simulink model "ADCS_Software_v1"  (R2026a)
settings: Solver=FixedStepAuto  StopTime=Inf  FixedStep=0.05  MaxStep=0.1
model workspace (MAT data in the model file):
  I_RW : Simulink.Parameter (value not decoded)
  Sig : Simulink.Signal (value not decoded)
  h_max : Simulink.Parameter (value not decoded)
  k_desat : Simulink.Parameter (value not decoded)
  kd_detumble : Simulink.Parameter (value not decoded)
  kd_hold : Simulink.Parameter (value not decoded)
  kd_point : Simulink.Parameter (value not decoded)
  kd_slew_fast : Simulink.Parameter (value not decoded)
  kd_slew_slow : Simulink.Parameter (value not decoded)
  kd_spin : Simulink.Parameter (value not decoded)
  kp_hold : Simulink.Parameter (value not decoded)
  kp_point : Simulink.Parameter (value not decoded)
  kp_slew_fast : Simulink.Parameter (value not decoded)
  kp_slew_slow : Simulink.Parameter (value not decoded)
  kp_spin : Simulink.Parameter (value not decoded)
values from neighbouring files (symbols this model uses):
  h_max = 1.47    [parameters.m]
  I_RW = 1    [parameters.m]
  k_desat = 1    [parameters.m]
  kd_detumble = 1    [parameters.m]
  kd_point = 20    [parameters.m]
  kd_spin = 0    [parameters.m]
  kp_point = 2    [parameters.m]
  kp_spin = 1    [parameters.m]
  omega_thr = 0.1    [parameters.m]
  omega_zero = 0.01    [parameters.m]
libraries: matrix_library x10, simulink x4, aerolibutil x2
(part 2 of 2)

== matlab function ADCS_Software_v1/Subsystem3/Controller/Control Algorithms/RW Torque Commands/OPTICAL/MATLAB Function2 ==
  data: y_cm output; x_cm output; u input
function [y_cm,x_cm] = fcn(u)
% u(u>5) = uint8(255);
% y = zeros(size(u,1),size(u,2));
% for i = 1:size(u,1)
%     for j = 1:size(u,2)
%         y(i,j) = double(max(u(i,j,:)));
%     end
% end
% S = sum(sum(y));
% if S == 0
%     x_cm = 0;
%     y_cm = 0;
% else
%     x_cm = sum(sum(y.*(1:size(y,2)),2))/S - size(y,2)/2;
%     y_cm = sum(sum(y.*(1:size(y,1))',1))/S- size(y,1)/2;
% end

y = double(max(u, [], 3));

% Binary foreground
bw = y > 5;

% Connected components
CC = bwconncomp(bw, 8);

if CC.NumObjects == 0
    x_cm = 0;
    y_cm = 0;
else
    % Calculate area of every component
    areas = cellfun(@numel, CC.PixelIdxList);

    % Largest connected component = satellite
    [~, idx] = max(areas);

    satelliteMask = false(size(bw));
    satelliteMask(CC.PixelIdxList{idx}) = true;

    % Geometric centroid
    [r, c] = find(satelliteMask);

    x_cm = mean(c) - size(y,2)/2;
    y_cm = mean(r) - size(y,1)/2;
end

== matlab function ADCS_Software_v1/MATLAB Function ==
  data: image input; quaternion output; use_previous input; previous_quaternion input; attitude_deg output; valid output; info output
function [quaternion, attitude_deg, valid, info] = startracker_sl(image, use_previous, previous_quaternion)
%#codegen
%STARTRACKER_SL  startracker.m for a Simulink MATLAB Function block / C code.
%
%   [q, attitude_deg, valid, info] = STARTRACKER_SL(image, use_previous, previous_quaternion)
%
%   Same algorithm, catalogue and conventions as startracker.m, rewritten so
%   MATLAB Coder / Simulink Coder can generate C from it:
%
%     * the catalogue comes from catalogue.mat through coder.load, so it is
%       compiled into the C code as constant data -- no file I/O at run time.
%       Make catalogue.mat with convert_catalogue.m and keep it on the MATLAB
%       path (or in the model's folder) when the model is built.
%     * every array has a fixed size: no growing arrays, cells, strings,
%       graph/conncomp, accumarray, sortrows, unique, intersect or eig.
%     * the info struct is replaced by a fixed 1x8 numeric vector.
%
%   Inputs:
%
%     image                2-D uint8 frame (1024x1024 for the shipped camera).
%                          Must be fixed-size in the Simulink block.
%     use_previous         0 = lost in space, 1 = tracking around input 3
%     previous_quaternion  1x4 or 4x1 [w x y z], scalar-first, the previous
%                          boresight (camera) attitude -- e.g. the fed-back
%                          output of this block
%
%   Outputs:
%
%     quaternion    1x4 [w x y z], scalar-first, the boresight (camera)
%                   attitude [CN]: the rotation carrying inertial (J2000)
%                   components into camera components, with +Z_C the
%                   boresight, +X_C image columns, +Y_C image rows.  NaN when
%                   not solved.
%     attitude_deg  1x3 boresight RA, Dec and roll about the boresight, in
%                   degrees (roll 0 = celestial north toward image row 0).
%                   NaN when not solved.
%     valid         true when quaternion is a fix
%     info          1x8 double:
%                     1  mode            0 = lost in space, 1 = tracking
%                     2  nDetections     stars detected in the frame
%                     3  nConsidered     brightest detections used (<= 15)
%                     4  nMatched        stars used in the final QUEST
%                     5  nSearched       catalogue stars searched
%                     6  residualArcsec  mean residual, NaN when not solved
%                     7  reasonCode      0 solved
%                                        1 too few detections
%                                        2 fewer than four detections
%                                        3 triad budget exhausted
%                                        4 no confirmed pyramid
%                     8  fallbackCode    0 none
%                                        1 previous quaternion not finite / zero
%                                        2 tracking found no match
%                                        3 previous boresight in no region
%
%   VALID = FALSE IS AN ANSWER: hold the last good attitude when it is false.
%
%   In the MATLAB Function block just call this function:
%
%       function [q, att, valid, info] = fcn(image, use_previous, previous_q)
%       [q, att, valid, info] = startracker_sl(image, use_previous, previous_q);
%
%   or paste this whole file into the block (rename the first function to
%   fcn, or keep its name -- the block uses the first function).

q_BC  = [0, 0, 0.707106781186548, 0.707106781186548];   % camera mounting (from DCM_CB')
q_sky = [0.707106781186548, 0, 0, 0.707106781186548];   % Vizard sky offset (from R_sky) - SIM ONLY


% In generated code (Simulink, C) coder.load runs at compile time: the
% catalogue becomes static const data, nothing is loaded at run time.  Run as
% plain MATLAB, coder.load would read the file on every call, so it is cached.
if coder.target('MATLAB')
    catalog = cachedCatalogue();
else
    catalog = coder.load('catalogue.mat');
end

% Settings, identical to startracker.m.
kDetections = 15;        % brightest detections handed to identification
minMatched = 4;          % fewest correspondences worth a quaternion
maxTriads = 400;         % triad budget before giving up
expandRadiusPx = 3.0;    % match growth radius
trackRings = 1;          % how far the tracking region walk spreads

quaternion = NaN(1, 4);
attitude_deg = NaN(1, 3);
valid = false;
info = zeros(1, 8);
info(6) = NaN;

tolerance = 3.5 * sqrt(2) * catalog.centroidSigmaPx / catalog.focalLengthPx;

% ---------------------------------------------------------------- detect ---
if isa(image, 'uint8')
    frame = image;
else
    frame = uint8(image);
end
[u, v, nTop, nDetections] = detectStars(frame, catalog.detectionSigma, kDetections);
info(2) = nDetections;

if nDetections < minMatched
    info(7) = 1;
    return;
end

n = nTop;
body = pixelToCamera(catalog, u, v, n);   % kDetections x 3, rows 1..n valid
info(3) = n;

% -------------------------------------------------------------- identify ---
priorMask = false(size(catalog.regionCentres, 1), 1);
havePrior = false;
if use_previous ~= 0
    qPrev = double(previous_quaternion(:)');
    if ~all(isfinite(qPrev)) || norm(qPrev) == 0
        info(8) = 1;
    else
        previousDcm = quatToDcm(qPrev);
        [priorMask, nPrior] = regionsContaining(catalog, previousDcm(3, :), priorMask, false);
        if nPrior > 0
            havePrior = true;
        else
            info(8) = 3;
        end
    end
end

tracking = false;
success = false;
detectionIndex = zeros(1, 4);
catalogueIndex = zeros(1, 4);
reasonCode = 4;

if havePrior
    searchRegions = regionNeighbourhood(catalog, priorMask, trackRings);
    starMask = subsetMask(catalog, searchRegions);
    [success, detectionIndex, catalogueIndex, reasonCode] = ...
        identifyPyramid(body, n, catalog, tolerance, maxTriads, starMask);
    if success
        tracking = true;
        info(1) = 1;
        info(5) = sum(starMask);
    else
        info(8) = 2;
    end
end

if ~success
    starMask = true(size(catalog.vectors, 1), 1);       % whole catalogue
    [success, detectionIndex, catalogueIndex, reasonCode] = ...
        identifyPyramid(body, n, catalog, tolerance, maxTriads, starMask);
    info(1) = 0;
    info(5) = catalog.nStars;
end

info(7) = reasonCode;
if ~success
    return;
end

% ---------------------------------------------------------------- attitude -
% Provisional attitude from the confirmed pyramid, then grow the match set.
provisional = quatToDcm(questQuaternion(body, detectionIndex, ...
                                        catalog.vectors, catalogueIndex, 4));

poolMask = true(size(catalog.vectors, 1), 1);
if tracking
    [regionIds, ~] = regionsContaining(catalog, provisional(3, :), priorMask, true);
    poolMask = subsetMask(catalog, regionNeighbourhood(catalog, regionIds, 1));
    if ~any(poolMask)
        poolMask(:) = true;   % startracker.m: empty candidates = whole catalogue
    end
end

expandTolerance = expandRadiusPx / catalog.focalLengthPx;
[expDet, expCat, nExp] = expandMatches(provisional, body, n, catalog, ...
                                       expandTolerance, poolMask);

if nExp >= minMatched
    matchedDet = expDet;
    matchedCat = expCat;
    nMatched = nExp;
else
    matchedDet = zeros(kDetections, 1);
    matchedCat = zeros(kDetections, 1);
    matchedDet(1:4) = detectionIndex;
    matchedCat(1:4) = catalogueIndex;
    nMatched = 4;
end

q = questQuaternion(body, matchedDet, catalog.vectors, matchedCat, nMatched);
q = quatmultiply(q_sky,quatmultiply(q,q_BC));
dcm = quatToDcm(q);
[ra, dec, roll] = dcmToRadecRoll(dcm);
residualSum = 0;
for m = 1:nMatched
    b = body(matchedDet(m), :);
    p = (dcm * catalog.vectors(matchedCat(m), :)')';
    residualSum = residualSum + atan2(norm(cross(b, p)), dot(b, p));
end

quaternion = q;
attitude_deg = [ra, dec, roll];
valid = true;
info(4) = nMatched;
info(6) = (residualSum / nMatched) * 180 / pi * 3600;
end


%% ======================================================== index queries ===

function [start, stop] = pairSpan(catalog, low, high)
%PAIRSPAN  Index range of the pair table that may hold separations in [low, high].
n = catalog.nPairs;
start = 0;
stop = 0;
if n < 2 || high < catalog.pairSep(1) || low > catalog.pairSep(n)
    return;
end
jLow = min(max(floor((low - catalog.kIntercept) / catalog.kSlope), 1), n);
jHigh = min(max(ceil((high - catalog.kIntercept) / catalog.kSlope), 1), n);
start = double(catalog.kVector(jLow));
stop = double(catalog.kVector(jHigh));
end


function [out, count] = neighbours(catalog, star, separation, tolerance, mask)
%NEIGHBOURS  Catalogue stars at SEPARATION +/- TOLERANCE from STAR, in mask.
out = zeros(maxNeighbours(), 1);
count = 0;
first = double(catalog.neighStart(star)) + 1;
last = double(catalog.neighStart(star + 1));
low = separation - tolerance;
high = separation + tolerance;
for s = first:last
    sep = catalog.neighSep(s);
    if sep >= low && sep <= high
        id = double(catalog.neighId(s));
        if mask(id)
            count = count + 1;
            out(count) = id;
        end
    end
end
end


function [common, nCommon, mark] = intersectIds(a, nA, b, nB, mark)
%INTERSECTIDS  Sorted unique values present in both lists (like intersect).
%   MARK is an all-false scratch vector over the stars; it is returned clean.
common = zeros(size(b));
nCommon = 0;
for i = 1:nA
    mark(a(i)) = true;
end
for i = 1:nB
    id = b(i);
    if mark(id)
        nCommon = nCommon + 1;
        common(nCommon) = id;
        mark(id) = false;          % de-duplicates
    end
end
for i = 1:nA
    mark(a(i)) = false;
end
common = insertionSort(common, nCommon);
end


function x = insertionSort(x, n)
%INSERTIONSORT  Sort x(1:n) ascending in place.
for i = 2:n
    key = x(i);
    j = i - 1;
    while j >= 1 && x(j) > key
        x(j + 1) = x(j);
        j = j - 1;
    end
    x(j + 1) = key;
end
end


%% ======================================================== regions =========

function [found, nFound] = regionsContaining(catalog, direction, startMask, useStart)
%REGIONSCONTAINING  Logical mask of every region whose cap contains DIRECTION.
%   With USESTART the search walks the adjacency graph from the regions in
%   STARTMASK; the answer is exact either way.
found = false(size(catalog.regionCentres, 1), 1);
nFound = 0;
if ~catalog.hasRegions
    return;
end
direction = direction(:);
cosRadius = catalog.regionCosRadius;

if useStart && any(startMask)
    best = -Inf;
    current = 0;
    for r = 1:catalog.nRegions
        if startMask(r)
            d = catalog.regionCentres(r, :) * direction;
            if d > best
                best = d;
                current = r;
            end
        end
    end

    while best < cosRadius
        first = double(catalog.regionAdjStart(current)) + 1;
        last = double(catalog.regionAdjStart(current + 1));
        value = -Inf;
        at = 0;
        for s = first:last
            id = double(catalog.regionAdjId(s));
            d = catalog.regionCentres(id, :) * direction;
            if d > value
                value = d;
                at = id;
            end
        end
        if at == 0 || value <= best
            break;                    % stalled: fall through to the full scan
        end
        current = at;
        best = value;
    end

    if best >= cosRadius
        found(current) = true;
        first = double(catalog.regionAdjStart(current)) + 1;
        last = double(catalog.regionAdjStart(current + 1));
        for s = first:last
            id = double(catalog.regionAdjId(s));
            if catalog.regionCentres(id, :) * direction >= cosRadius
                found(id) = true;
            end
        end
        nFound = sum(found);
        return;
    end
end

for r = 1:catalog.nRegions
    if catalog.regionCentres(r, :) * direction >= cosRadius
        found(r) = true;
    end
end
nFound = sum(found);
end


function selected = regionNeighbourhood(catalog, regionMask, rings)
%REGIONNEIGHBOURHOOD  REGIONMASK plus every region within RINGS adjacency steps.
selected = regionMask;
frontier = regionMask;
for ring = 1:max(0, rings)
    reached = false(size(catalog.regionCentres, 1), 1);
    for r = 1:catalog.nRegions
        if frontier(r)
            first = double(catalog.regionAdjStart(r)) + 1;
            last = double(catalog.regionAdjStart(r + 1));
            for s = first:last
                id = double(catalog.regionAdjId(s));
                if ~selected(id)
                    reached(id) = true;
                end
            end
        end
    end
    if ~any(reached)
        break;
    end
    selected = selected | reached;
    frontier = reached;
end
end


function mask = subsetMask(catalog, regionMask)
%SUBSETMASK  Logical vector of the stars inside the regions of REGIONMASK.
mask = false(size(catalog.vectors, 1), 1);
for r = 1:catalog.nRegions
    if regionMask(r)
        first = double(catalog.regionMemStart(r)) + 1;
        last = double(catalog.regionMemStart(r + 1));
        for s = first:last
            mask(catalog.regionMemStar(s)) = true;
        end
    end
end
end


%% ======================================================== detection ======

function [u, v, nTop, nDetections] = detectStars(frame, thresholdSigma, kMax)
%DETECTSTARS  Background, threshold, 8-connected segmentation, centroiding.
%
%   Returns only the KMAX brightest detections, sorted by flux (descending,
%   stable -- the same order startracker.m's sort gives), plus the total
%   count.  Components are found by flood fill in column-major scan order,
%   which is the order conncomp numbers them in startracker.m.
%   Pixel (row i, column j) has its centre at (u, v) = (j - 0.5, i - 0.5).

minPixels = 2;
u = zeros(kMax, 1);
v = zeros(kMax, 1);
flux = zeros(kMax, 1);
nTop = 0;
nDetections = 0;

[background, noise] = backgroundAndNoise(frame);
threshold = floor(background + thresholdSigma * noise) + 1;
if threshold > 255
    return;
end

height = size(frame, 1);
width = size(frame, 2);
visited = false(height, width);
stack = zeros(height * width, 1, 'int32');

for col = 1:width
    for row = 1:height
        if visited(row, col) || double(frame(row, col)) < threshold
            continue;
        end

        % ---- flood fill one component ----
        visited(row, col) = true;
        top = 1;
        stack(1) = int32((col - 1) * height + row);
        total = 0;
        sumU = 0;
        sumV = 0;
        count = 0;
        while top > 0
            p = double(stack(top)) - 1;
            top = top - 1;
            pr = mod(p, height) + 1;
            pc = floor(p / height) + 1;

            % A pixel exactly at the threshold can carry a non-positive weight;
            % it still belongs to the component, it just does not pull.
            w = double(frame(pr, pc)) - background;
            total = total + w;
            sumU = sumU + w * (pc - 0.5);
            sumV = sumV + w * (pr - 0.5);
            count = count + 1;

            for dc = -1:1
                nc = pc + dc;
                if nc < 1 || nc > width
                    continue;
                end
                for dr = -1:1
                    nr = pr + dr;
                    if nr < 1 || nr > height || (dr == 0 && dc == 0)
                        continue;
                    end
                    if ~visited(nr, nc) && double(frame(nr, nc)) >= threshold
                        visited(nr, nc) = true;
                        top = top + 1;
                        stack(top) = int32((nc - 1) * height + nr);
                    end
                end
            end
        end

        if count < minPixels || total <= 0
            continue;
        end
        nDetections = nDetections + 1;

        % ---- keep the kMax brightest, stable for equal flux ----
        pos = nTop + 1;
        for t = 1:nTop
            if flux(t) < total
                pos = t;
                break;
            end
        end
        if pos > kMax
            continue;
        end
        last = min(nTop, kMax - 1);
        for t = last:-1:pos
            u(t + 1) = u(t);
            v(t + 1) = v(t);
            flux(t + 1) = flux(t);
        end
        u(pos) = sumU / total;
        v(pos) = sumV / total;
        flux(pos) = total;
        nTop = min(nTop + 1, kMax);
    end
end
end


function [background, noise] = backgroundAndNoise(frame)
%BACKGROUNDANDNOISE  Robust level (median) and noise (MAD) from a histogram.
histogram = zeros(256, 1);
total = numel(frame);
for p = 1:total
    b = double(frame(p)) + 1;
    histogram(b) = histogram(b) + 1;
end
if total == 0
    background = 0;
    noise = 1;
    return;
end

half = floor(total / 2);
background = 0;
running = 0;
for b = 1:256
    running = running + histogram(b);
    if running > half
        background = b - 1;
        break;
    end
end

deviations = zeros(256, 1);
for b = 0:255
    d = abs(b - background) + 1;
    deviations(d) = deviations(d) + histogram(b + 1);
end
mad = 0;
running = 0;
for d = 1:256
    running = running + deviations(d);
    if running > half
        mad = d - 1;
        break;
    end
end

noise = max(1.4826 * mad, 0.5);
end


%% ======================================================== identification ==

function [success, detectionIndex, catalogueIndex, reasonCode] = ...
    identifyPyramid(body, n, catalog, tolerance, maxTriads, mask)
%IDENTIFYPYRAMID  Match a pyramid: a confirmed triangle plus a fourth star.
%   A solution is returned only when the confirmed assignment is unique.
success = false;
detectionIndex = zeros(1, 4);
catalogueIndex = zeros(1, 4);

if n < 4
    reasonCode = 2;
    return;
end

theta = angularSeparations(body, n);
mark = false(size(catalog.vectors, 1), 1);
triads = 0;

% (i, j, k) by increasing index gaps (Mortari), as startracker.m triadOrder.
for gapJ = 1:n - 2
    for gapK = 1:n - gapJ - 1
        for i = 1:n - gapJ - gapK
            j = i + gapJ;
            k = j + gapK;

            if triads >= maxTriads
                reasonCode = 3;
                return;
            end
            triads = triads + 1;

            [found, nFound, mark] = candidateTriangles(catalog, theta(i, j), ...
                theta(i, k), theta(j, k), tolerance, mask, mark);
            if nFound == 0
                continue;
            end

            for r = 1:n
                if r == i || r == j || r == k
                    continue;
                end

                nConfirmed = 0;
                firstConfirmed = zeros(1, 4);
                for c = 1:nFound
                    [fourth, nFourth, mark] = confirmFourth(catalog, found(c, :), ...
                        [theta(i, r), theta(j, r), theta(k, r)], tolerance, mask, mark);
                    for f = 1:nFourth
                        nConfirmed = nConfirmed + 1;
                        if nConfirmed == 1
                            firstConfirmed = [found(c, :), fourth(f)];
                        else
                            break;
                        end
                    end
                    if nConfirmed > 1
                        break;
                    end
                end

                if nConfirmed == 1
                    success = true;
                    detectionIndex = [i, j, k, r];
                    catalogueIndex = firstConfirmed;
                    reasonCode = 0;
                    return;
                end
            end
        end
    end
end

reasonCode = 4;
end


function [found, nFound, mark] = candidateTriangles(catalog, thetaIJ, thetaIK, ...
                                                    thetaJK, tolerance, mask, mark)
%CANDIDATETRIANGLES  Catalogue triples whose three separations match the input.
limit = 5000;
found = zeros(limit, 3);
nFound = 0;

low = thetaIJ - tolerance;
high = thetaIJ + tolerance;
[start, stop] = pairSpan(catalog, low, high);

for p = start + 1:stop
    sep = catalog.pairSep(p);
    if sep < low || sep > high
        continue;
    end
    pa = double(catalog.pairA(p));
    pb = double(catalog.pairB(p));
    if ~mask(pa) || ~mask(pb)
        continue;
    end

    % Each pair is stored once: detection i may sit at either end.
    for e = 1:2
        if e == 1
            a = pa;
            b = pb;
        else
            a = pb;
            b = pa;
        end

        [fromA, nA] = neighbours(catalog, a, thetaIK, tolerance, mask);
        if nA == 0
            continue;
        end
        [fromB, nB] = neighbours(catalog, b, thetaJK, tolerance, mask);
        if nB == 0
            continue;
        end

        [common, nCommon, mark] = intersectIds(fromA, nA, fromB, nB, mark);
        for t = 1:nCommon
            c = common(t);
            if c ~= a && c ~= b
                nFound = nFound + 1;
                found(nFound, :) = [a, b, c];
                if nFound >= limit
                    return;
                end
            end
        end
    end
end
end


function [out, nOut, mark] = confirmFourth(catalog, triangle, thetaR, tolerance, mask, mark)
%CONFIRMFOURTH  Catalogue stars at the right distance from all three vertices,
%   sorted ascending, excluding the triangle itself.
out = zeros(maxNeighbours(), 1);
nOut = 0;

[fromA, nA] = neighbours(catalog, triangle(1), thetaR(1), tolerance, mask);
if nA == 0
    return;
end
[fromB, nB] = neighbours(catalog, triangle(2), thetaR(2), tolerance, mask);
if nB == 0
    return;
end
[common, nCommon, mark] = intersectIds(fromA, nA, fromB, nB, mark);
if nCommon == 0
    return;
end
[fromC, nC] = neighbours(catalog, triangle(3), thetaR(3), tolerance, mask);
if nC == 0
    return;
end
[both, nBoth, mark] = intersectIds(common, nCommon, fromC, nC, mark);

for t = 1:nBoth
    id = both(t);
    if id ~= triangle(1) && id ~= triangle(2) && id ~= triangle(3)
        nOut = nOut + 1;
        out(nOut) = id;
    end
end
end


function theta = angularSeparations(body, n)
%ANGULARSEPARATIONS  Angles between every pair of body vectors, in radians,
%   through atan2(|a x b|, a . b), which keeps small angles accurate.
theta = zeros(size(body, 1));
for i = 1:n - 1
    for j = i + 1:n
        angle = atan2(norm(cross(body(i, :), body(j, :))), ...
                      dot(body(i, :), body(j, :)));
        theta(i, j) = angle;
        theta(j, i) = angle;
    end
end
end


function [detectionIndex, catalogueIndex, nOut] = expandMatches(dcm, body, n, ...
                                                    catalog, tolerance, poolMask)
%EXPANDMATCHES  Grow a confirmed solution by matching the remaining detections.
%   A detection is accepted only when its nearest catalogue star is inside
%   tolerance and no other catalogue star is; a catalogue star claimed by two
%   detections is dropped.
kMax = size(body, 1);
detectionIndex = zeros(kMax, 1);
catalogueIndex = zeros(kMax, 1);
nOut = 0;

cosTolerance = cos(tolerance);
boresight = dcm(3, :)';
cosField = cos(catalog.maxSeparationRad / 2 + 0.02);

% Cull to the stars that can land on the detector, predicted into body frame.
pool = zeros(size(catalog.vectors, 1), 1);
predicted = zeros(size(catalog.vectors, 1), 3);
nPool = 0;
for s = 1:catalog.nStars
    if poolMask(s) && catalog.vectors(s, :) * boresight >= cosField
        nPool = nPool + 1;
        pool(nPool) = s;
        predicted(nPool, :) = (dcm * catalog.vectors(s, :)')';
    end
end
if nPool == 0
    return;
end

nAccepted = 0;
accDet = zeros(kMax, 1);
accCat = zeros(kMax, 1);
for d = 1:n
    best = -Inf;
    bestAt = 0;
    second = -2;
    for s = 1:nPool
        sim = body(d, :) * predicted(s, :)';
        if sim > best
            if bestAt > 0
                second = best;
            end
            best = sim;
            bestAt = s;
        elseif sim > second
            second = sim;
        end
    end
    if best >= cosTolerance && second < cosTolerance
        nAccepted = nAccepted + 1;
        accDet(nAccepted) = d;
        accCat(nAccepted) = pool(bestAt);
    end
end

for a = 1:nAccepted
    claimedTwice = false;
    for b = 1:nAccepted
        if b ~= a && accCat(b) == accCat(a)
            claimedTwice = true;
            break;
        end
    end
    if ~claimedTwice
        nOut = nOut + 1;
        detectionIndex(nOut) = accDet(a);
        catalogueIndex(nOut) = accCat(a);
    end
end
end


%% ======================================================== attitude =======

function q = questQuaternion(body, detectionIndex, vectors, catalogueIndex, m)
%QUESTQUATERNION  Optimal attitude quaternion [w x y z], scalar-first, [CN] (camera frame).
%   Largest-eigenvalue eigenvector of Davenport's K matrix; the 4x4 symmetric
%   eigenproblem is solved by Jacobi rotations (eig is avoided because its
%   generated code returns complex results for real input).
profile = zeros(3);
for i = 1:m
    profile = profile + body(detectionIndex(i), :)' * vectors(catalogueIndex(i), :);
end

sigma = trace(profile);
axis = [profile(2, 3) - profile(3, 2);
        profile(3, 1) - profile(1, 3);
        profile(1, 2) - profile(2, 1)];

K = zeros(4);
K(1:3, 1:3) = profile + profile' - sigma * eye(3);
K(1:3, 4) = axis;
K(4, 1:3) = axis';
K(4, 4) = sigma;

[values, vecs] = jacobiEigen4(K);
largest = 1;
for i = 2:4
    if values(i) > values(largest)
        largest = i;
    end
end
w = vecs(:, largest);

q = [w(4), w(1), w(2), w(3)];
q = q / norm(q);
if q(1) < 0
    q = -q;                       % one quaternion per attitude, not two
end
end


function [values, V] = jacobiEigen4(A)
%JACOBIEIGEN4  Eigen-decomposition of a real symmetric 4x4 matrix by cyclic
%   Jacobi rotations.  values(i) belongs to column V(:, i).
V = eye(4);
scale = max(norm(A, 'fro'), realmin);
for sweep = 1:50
    off = 0;
    for p = 1:3
        for r = p + 1:4
            off = off + A(p, r)^2;
        end
    end
    if sqrt(off) <= 1e-15 * scale
        break;
    end
    for p = 1:3
        for r = p + 1:4
            if A(p, r) == 0
                continue;
            end
            tau = (A(r, r) - A(p, p)) / (2 * A(p, r));
            if tau >= 0
                t = 1 / (tau + sqrt(1 + tau^2));
            else
                t = -1 / (-tau + sqrt(1 + tau^2));
            end
            c = 1 / sqrt(1 + t^2);
            s = t * c;
            G = eye(4);
            G(p, p) = c;
            G(r, r) = c;
            G(p, r) = s;
            G(r, p) = -s;
            A = G' * A * G;
            A(p, r) = 0;
            A(r, p) = 0;
            V = V * G;
        end
    end
end
values = diag(A);
end


function dcm = quatToDcm(q)
%QUATTODCM  Scalar-first quaternion to the direction cosine matrix [CN].
q = q(:)' / norm(q);
q0 = q(1); q1 = q(2); q2 = q(3); q3 = q(4);

dcm = [q0^2 + q1^2 - q2^2 - q3^2,  2 * (q1 * q2 + q0 * q3),  2 * (q1 * q3 - q0 * q2);
       2 * (q1 * q2 - q0 * q3),  q0^2 - q1^2 + q2^2 - q3^2,  2 * (q2 * q3 + q0 * q1);
       2 * (q1 * q3 + q0 * q2),  2 * (q2 * q3 - q0 * q1),  q0^2 - q1^2 - q2^2 + q3^2];
end


function [ra, dec, roll] = dcmToRadecRoll(dcm)
%DCMTORADECROLL  [CN] to boresight RA, Dec and roll in degrees (roll 0 = north up).
xC = dcm(1, :);
zC = dcm(3, :);

ra = mod(atan2(zC(2), zC(1)), 2 * pi);
dec = asin(max(-1, min(1, zC(3))));

reference = [0, 0, 1];
y0 = reference - dot(reference, zC) * zC;
if norm(y0) < 1e-8
    reference = [1, 0, 0];        % the boresight is on the pole
    y0 = reference - dot(reference, zC) * zC;
end
y0 = -y0 / norm(y0);
x0 = cross(y0, zC);
roll = mod(atan2(dot(xC, y0), dot(xC, x0)), 2 * pi);

ra = ra * 180 / pi;
dec = dec * 180 / pi;
roll = roll * 180 / pi;
end


function body = pixelToCamera(catalog, u, v, n)
%PIXELTOCAMERA  Pixel coordinates to unit camera-frame vectors (ideal pinhole).
%   +Z boresight, +X along columns (u, right), +Y along rows (v, down).
body = zeros(numel(u), 3);
for i = 1:n
    x = (u(i) - catalog.principalPointPx(1)) / catalog.focalLengthPx;
    y = (v(i) - catalog.principalPointPx(2)) / catalog.focalLengthPx;
    len = sqrt(x^2 + y^2 + 1);
    body(i, :) = [x, y, 1] / len;
end
end


function n = maxNeighbours()
%MAXNEIGHBOURS  Longest per-star neighbour list, as a compile-time constant
%   (it sizes the fixed neighbour buffers).
limits = coder.load('catalogue.mat', 'maxNeighbours');
n = limits.maxNeighbours;
end


function catalog = cachedCatalogue()
%CACHEDCATALOGUE  MATLAB-only: read catalogue.mat once and keep it.
%   Never compiled -- the caller only reaches it when coder.target('MATLAB').
%   Run `clear startracker_sl` after regenerating catalogue.mat.
persistent cached
if isempty(cached)
    cached = load('catalogue.mat');
end
catalog = cached;
end

== stateflow chart ADCS_Software_v1/Subsystem3/Mode manager/Status_Manager ==
  state STATUS
    during:
    mode_degraded = (actual_ephem ~= desired_ephem) || (actual_ads ~= desired_ads) || (actual_frame ~= desired_frame) || (actual_acs ~= desired_acs);
  (default) -> STATUS
  data: desired_ephem input uint8; desired_ads input uint8; desired_frame input uint8; desired_acs input uint8; actual_ephem input uint8; actual_ads input uint8; actual_frame input uint8; actual_acs input uint8; mode_degraded output boolean =0

== stateflow chart ADCS_Software_v1/Subsystem3/Mode manager/Mode Manager/Ephemeris_Manager ==
  state EPHEM_IDLE
    entry:
    actual_ephem = uint8(0);
  state EPHEM_GPS
    entry:
    actual_ephem = uint8(2);
  state EPHEM_TLE
    entry:
    actual_ephem = uint8(1);
  EPHEM_GPS -> EPHEM_IDLE [order 1] : [desired_ephem == uint8(0)]
  EPHEM_IDLE -> EPHEM_GPS [order 2] : [desired_ephem == uint8(2)...
      |  && gps_valid]
  (default) -> EPHEM_IDLE
  EPHEM_IDLE -> EPHEM_TLE [order 1] : [desired_ephem == uint8(1) ||...
      |  (desired_ephem == uint8(2) &&...
      |  ~gps_valid && ~tle_error_high)]
  EPHEM_TLE -> EPHEM_IDLE [order 1] : [desired_ephem == uint8(0)...
      |  || tle_error_high]
  EPHEM_GPS -> EPHEM_TLE [order 2] : [desired_ephem == uint8(1) ||...
      |  ~gps_valid]
  EPHEM_TLE -> EPHEM_GPS [order 2] : [desired_ephem == uint8(2) && gps_valid]
  data: desired_ephem input uint8; gps_valid input boolean; tle_error_high input boolean; actual_ephem output uint8 =0

== stateflow chart ADCS_Software_v1/Subsystem3/Mode manager/Mode Manager/ADS_Manager ==
  state ADS_IDLE
    entry:
    actual_ads = uint8(0);
  state ADS_UKF_FINE
    entry:
    actual_ads = uint8(2);
  state ADS_UKF_COARSE
    entry:
    actual_ads = uint8(1);
  ADS_UKF_FINE -> ADS_IDLE [order 2] : [desired_ads == uint8(0) || ads_fault]
  ADS_IDLE -> ADS_UKF_FINE [order 2] : [desired_ads == uint8(2) &&...
      |  ads_fine_allowed && ~ads_fault]
  (default) -> ADS_IDLE
  ADS_UKF_COARSE -> ADS_IDLE [order 1] : [desired_ads == uint8(0) || ads_fault]
  ADS_IDLE -> ADS_UKF_COARSE [order 1] : [desired_ads == uint8(1) ||...
      |  (desired_ads == uint8(2) &&...
      |  ~ads_fine_allowed)]
  ADS_UKF_FINE -> ADS_UKF_COARSE [order 1] : [desired_ads == uint8(1) ||...
      |  ~ads_fine_allowed]
  ADS_UKF_COARSE -> ADS_UKF_FINE [order 2] : [desired_ads == uint8(2) &&...
      |  ads_fine_allowed && ~ads_fault]
  data: desired_ads input uint8; ads_fine_allowed input boolean; ads_fault input boolean; actual_ads output uint8 =0

== stateflow chart ADCS_Software_v1/Subsystem3/Mode manager/Mode Manager/Mission_Mode_Manager ==
  state M_DETUMBLE
    entry:
    desired_ephem = uint8(0);
    desired_ads = uint8(1);
    desired_frame = uint8(0);
    desired_acs = uint8(1);
    %desired_actuator = uint8(3);
  state M_SAFE_SUN
    entry:
    desired_ephem = uint8(0);
    desired_ads = uint8(0);
    desired_frame = uint8(0);
    desired_acs = uint8(6);
    %desired_actuator = uint8(2);
  state M_Y_SPIN
    entry:
    desired_ephem = uint8(2);
    desired_ads = uint8(1);
    desired_frame = uint8(1);
    desired_acs = uint8(3);
    %desired_actuator = uint8(2);
  state M_IDLE
    entry:
    desired_ephem = uint8(0);
    desired_ads = uint8(0);
    desired_frame = uint8(0);
    desired_acs = uint8(0);
    %desired_actuator = uint8(0);
  state M_MIN_DRAG
    entry:
    desired_ephem = uint8(2);
    desired_ads = uint8(2);
    desired_frame = uint8(5);
    desired_acs = uint8(2);
    %desired_actuator = uint8(2);
  state M_POINT_NADIR
    entry:
    desired_ephem = uint8(2);
    desired_ads = uint8(2);
    desired_frame = uint8(3);
    desired_acs = uint8(2);
    %desired_actuator = uint8(2);
  state M_MAX_DRAG
    entry:
    desired_ephem = uint8(2);
    desired_ads = uint8(2);
    desired_frame = uint8(5);
    desired_acs = uint8(2);
    %desired_actuator = uint8(2);
  state M_POINT_EARTH_TARGET
    entry:
    desired_ephem = uint8(2);
    desired_ads = uint8(2);
    desired_frame = uint8(4);
    desired_acs = uint8(2);
    %desired_actuator = uint8(2);
  state M_RAM
    entry:
    desired_ephem = uint8(2);
    desired_ads = uint8(2);
    desired_frame = uint8(5);
    desired_acs = uint8(2);
    %desired_actuator = uint8(2);
  state M_POINT_SUN
    entry:
    desired_ephem = uint8(2);
    desired_ads = uint8(2);
    desired_frame = uint8(2);
    desired_acs = uint8(2);
    %desired_actuator = uint8(2);
  state M_INTERSAT_TRACK
    entry:
    desired_ephem = uint8(2);
    desired_ads = uint8(2);
    desired_frame = uint8(2);
    desired_acs = uint8(5);
    %desired_actuator = uint8(2);
  M_DETUMBLE -> (junction 28) : [mission_cmd ~= uint8(1)]
  (junction 28) -> M_DETUMBLE [order 3] : [mission_cmd == uint8(1)]
  M_Y_SPIN -> (junction 28) : [mission_cmd ~= uint8(3)]
  M_SAFE_SUN -> (junction 28) : [mission_cmd ~= uint8(2)]
  (junction 28) -> M_SAFE_SUN [order 4] : [mission_cmd == uint8(2)]
  M_IDLE -> (junction 28) : [mission_cmd ~= uint8(0)]
  (default) -> M_IDLE
  (junction 28) -> M_IDLE [order 1] : [mission_cmd == uint8(0)]
  (junction 28) -> M_Y_SPIN [order 5] : [mission_cmd == uint8(3)]
  (junction 28) -> M_MIN_DRAG [order 11] : [mission_cmd == uint8(8)]
  M_MIN_DRAG -> (junction 28) : [mission_cmd ~= uint8(8)]
  (junction 28) -> M_POINT_NADIR [order 6] : [mission_cmd == uint8(4)]
  M_POINT_NADIR -> (junction 28) : [mission_cmd ~= uint8(4)]
  (junction 28) -> M_MAX_DRAG [order 2] : [mission_cmd == uint8(9)]
  M_MAX_DRAG -> (junction 28) : [mission_cmd ~= uint8(9)]
  (junction 28) -> M_POINT_EARTH_TARGET [order 8] : [mission_cmd == uint8(6)]
  (junction 28) -> M_POINT_SUN [order 7] : [mission_cmd == uint8(5)]
  M_POINT_EARTH_TARGET -> (junction 28) : [mission_cmd ~= uint8(6)]
  M_POINT_SUN -> (junction 28) : [mission_cmd ~= uint8(5)]
  (junction 28) -> M_INTERSAT_TRACK [order 9] : [mission_cmd == uint8(7)]
  (junction 28) -> M_RAM [order 10] : [mission_cmd == uint8(10)]
  M_INTERSAT_TRACK -> (junction 28) : [mission_cmd ~= uint8(7)]
  M_RAM -> (junction 28) : [mission_cmd ~= uint8(10)]
  data: mission_cmd input uint8; intersat_sensor_tracking input boolean; desired_ephem output uint8 =0; desired_ads output uint8 =0; desired_frame output uint8 =0; desired_acs output uint8 =0
